simulink model "PFC_DSFB"  (R2023b)
settings: Solver=VariableStepAuto  StartTime=0.0  StopTime=0.5  RelTol=1e-3
libraries: spsVoltageMeasurementLib x5, spsSeriesRLCBranchLib x3, spsCurrentMeasurementLib x3, spsDiodeLib x3, spsMosfetLib x2, spsACVoltageSourceLib x1, simulink x1, spsLinearTransformerLib x1, spsMeanLib x1, slpidlib x1, powerlib_extras x1, simulink_extras x1
settings Model: SimulationMode=accelerator  Creator=abc6820292  LastModifiedBy=Qu
settings DebuggingCC: UnconnectedInputMsg=warning  UnconnectedOutputMsg=warning  UnconnectedLineMsg=warning
settings ModelReferenceCC: EnableRefExpFcnMdlSchedulingChecks=on
settings RTWCC: DLArmComputeVersion=19.05

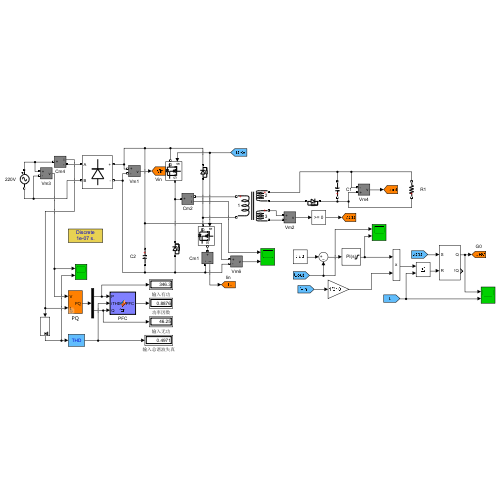
[thumbnail: Simulink's stored preview of the top-level diagram]
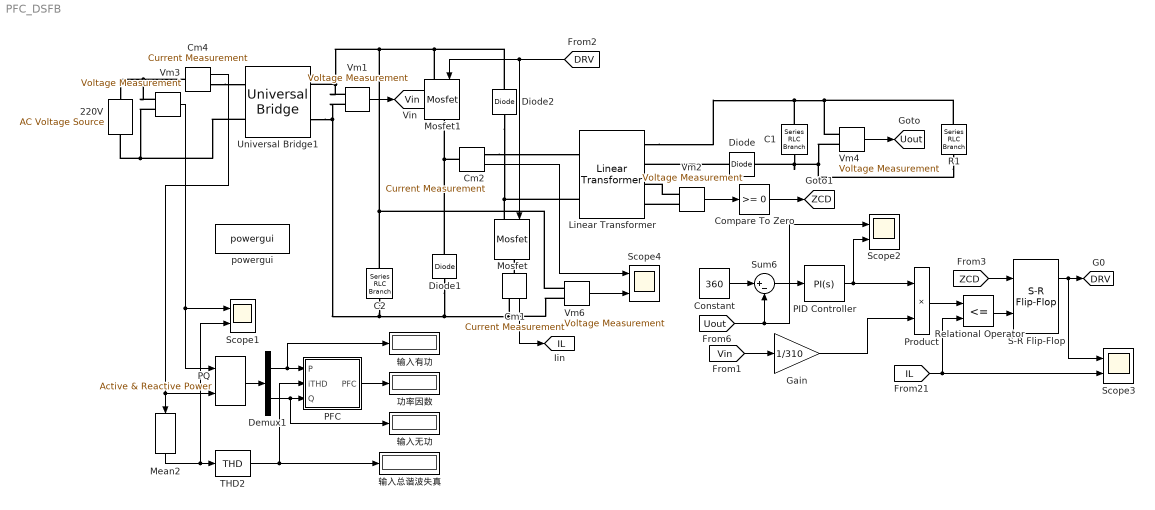
== system PFC_DSFB ==
  220V : spsACVoltageSourceLib/AC Voltage Source  Amplitude=220*1.414  Phase=0  Frequency=50  SampleTime=0  Measurements=None  BusType=swing  Pref=10e3  Qref=0  Qmin=-inf  Qmax=+inf
  C1 : spsSeriesRLCBranchLib/Series RLC Branch  LConnTagsString=__new0  RConnTagsString=__new0  BranchType=C  Resistance=10  Inductance=0  SetiL0=off  InitialCurrent=0  Capacitance=4e-4  Setx0=off  InitialVoltage=200  Measurements=None
  C2 : spsSeriesRLCBranchLib/Series RLC Branch  LConnTagsString=__new0  RConnTagsString=__new0  BranchType=C  Resistance=10  Inductance=0  SetiL0=off  InitialCurrent=0  Capacitance=5e-8  Setx0=off  InitialVoltage=200  Measurements=None
  Cm1 : spsCurrentMeasurementLib/Current Measurement  PhasorSimulation=off  OutputType=Complex  PSBequivalent=0
  Cm2 : spsCurrentMeasurementLib/Current Measurement  PhasorSimulation=off  OutputType=Complex  PSBequivalent=0
  Cm4 : spsCurrentMeasurementLib/Current Measurement  PhasorSimulation=off  OutputType=Complex  PSBequivalent=0
  Compare To Zero : simulink/Logic and Bit Operations/Compare To Zero  relop=>=  OutDataTypeStr=boolean
  Constant : Constant  Value=360
  Demux1 : Demux  Outputs=2
  Diode : spsDiodeLib/Diode  Ron=0.001  Lon=0  Vf=0.8  IC=0  UseSnubber=0  Rs=1e6  Cs=1e-9  Measurements=off
  Diode1 : spsDiodeLib/Diode  Ron=0.001  Lon=0  Vf=0.8  IC=0  UseSnubber=0  Rs=1e6  Cs=1e-9  Measurements=off
  Diode2 : spsDiodeLib/Diode  Ron=0.001  Lon=0  Vf=0.8  IC=0  UseSnubber=0  Rs=1e6  Cs=1e-9  Measurements=off
  Gain : Gain  Gain=1/310
  Linear Transformer : spsLinearTransformerLib/Linear Transformer  UNITS=SI  NominalPower=[600 60000]  winding1=[200 0.01 1e-6]  winding2=[500 0.01 1e-6]  ThreeWindings=on  winding3=[10 1 1e-6]  RmLm=[1e6 2e-4]  Measurements=None  DataType=on
  Mean2 : spsMeanLib/Mean  Freq=2000  Vinit=0  Ts=0
  Mosfet : spsMosfetLib/Mosfet  Ron=0.05  Lon=0  Rd=0.01  Vfd=0  IC=0  Rs=1e5  Cs=inf  Measurements=off
  Mosfet1 : spsMosfetLib/Mosfet  Ron=0.05  Lon=0  Rd=0.01  Vfd=0  IC=0  Rs=1e5  Cs=inf  Measurements=off
  PFC : MATLAB Function  TreatAsAtomicUnit=on
  PID Controller : slpidlib/PID Controller  Controller=PI  Form=Parallel  TimeDomain=Continuous-time  UseExternalTs=off  SampleTime=-1  IntegratorMethod=Forward Euler  FilterMethod=Forward Euler  ControllerParametersSource=internal  P=0.2  I=4  UseKiTs=off  D=0.001  N=100  UseFilter=on  TunerSelectOption=Transfer Function Based (PID Tuner App)  InitialConditionSource=internal  InitialConditionForIntegrator=0  InitialConditionForFilter=0  DifferentiatorICPrevScaledInput=0  ExternalReset=none  TrackingMode=off  Kt=1  LimitOutput=on  SatLimitsSource=internal  UpperSaturationLimit=30  LowerSaturationLimit=0  LinearizeAsGain=on  AntiWindupMode=clamping  Kb=1  LimitIntegrator=off  UpperIntegratorSaturationLimit=inf  LowerIntegratorSaturationLimit=-inf  POutMin=[]  POutMax=[]  IOutMin=[]  IOutMax=[]  DOutMin=[]  DOutMax=[]  NOutMin=[]  NOutMax=[]  SumOutMin=[]  SumOutMax=[]  SaturationOutMin=[]  SaturationOutMax=[]  PParamMin=[]  PParamMax=[]  IParamMin=[]  IParamMax=[]  DParamMin=[]  DParamMax=[]  NParamMin=[]  NParamMax=[]  KbParamMin=[]  KbParamMax=[]  KtParamMin=[]  KtParamMax=[]  KbOutMin=[]  KbOutMax=[]  KtOutMin=[]  KtOutMax=[]  IntegratorOutMin=[]  IntegratorOutMax=[]  FilterOutMin=[]  FilterOutMax=[]  SumI1OutMin=[]  SumI1OutMax=[]  SumI2OutMin=[]  SumI2OutMax=[]  SumI3OutMin=[]  SumI3OutMax=[]  SumI4OutMin=[]  SumI4OutMax=[]  SumDOutMin=[]  SumDOutMax=[]  DifferentiatorOutMin=[]  DifferentiatorOutMax=[]  FilterDiffOutCoefMin=[]  FilterDiffOutCoefMax=[]  ReciprocalOutMin=[]  ReciprocalOutMax=[]  SumDenOutMin=[]  SumDenOutMax=[]  SumNumOutMin=[]  SumNumOutMax=[]  DivideOutMin=[]  DivideOutMax=[]  UdiffTsProdOutMin=[]  UdiffTsProdOutMax=[]  NTsProdOutMin=[]  NTsProdOutMax=[]  UintegralTsProdOutMin=[]  UintegralTsProdOutMax=[]  UngainTsProdOutMin=[]  UngainTsProdOutMax=[]  ClampingZeroOutDataTypeStr=Inherit: Inherit via back propagation  ClampingZeroOutMin=[]  ClampingZeroOutMax=[]  FilterDenConstantOutDataTypeStr=Inherit: Inherit via back propagation  FilterDenConstantOutMin=[]  FilterDenConstantOutMax=[]  PCopyOutDataTypeStr=Inherit: Inherit via back propagation  PCopyOutMin=[]  PCopyOutMax=[]  NCopyOutDataTypeStr=Inherit: Inherit via back propagation  NCopyOutMin=[]  NCopyOutMax=[]  IntegratorContinuousStateAttributes=''  IntegratorStateMustResolveToSignalObject=off  IntegratorRTWStateStorageClass=Auto  FilterContinuousStateAttributes=''  FilterStateMustResolveToSignalObject=off  FilterRTWStateStorageClass=Auto  ParallelPVariant=InternalParameters  IdealPVariant=Disabled  IVariant=InternalParameters  DVariant=Disabled  IntegratorVariant=Continuous  SatVariant=Enabled  AWVariant=ContClampingParallel  PCopyVariant=Disabled  TRVariant=Disabled  FdbkBlocksVariant=Forward  IdealPFdbkVariant=Disabled  SatFdbkVariant=Disabled  DerivativeFilterVariant=Disabled  NVariant=Disabled  NCopyVariant=Disabled_SignalSpec  FilterICVariant=Disabled  IntegratorICVariant=InternalICs  ExternalResetVariant=Disabled  TRSumVariant=Passthrough  SumFdbkVariant=Disabled  SumVariant=Sum_PI  TsampFilterVariant=InternalTs  TsampNgainVariant=Passthrough  TsampIntegralVariant=Disabled_SignalSpec  ExternalSaturationOutDataTypeStr=Inherit: Same as second input
  PQ : powerlib_extras/Measurements/Active & Reactive Power  f1=50
  Product : Product
  R1 : spsSeriesRLCBranchLib/Series RLC Branch  LConnTagsString=__new0  RConnTagsString=__new0  BranchType=R  Resistance=220  Inductance=0  SetiL0=off  InitialCurrent=0  Capacitance=8e-3  Setx0=on  InitialVoltage=280  Measurements=None
  Relational Operator : RelationalOperator  Operator=<=  OutDataTypeStr=boolean  RndMeth=Simplest  InputSameDT=off
  S-R Flip-Flop : simulink_extras/Flip Flops/S-R Flip-Flop  initial_condition=0
  Scope{1..4} (4 alike) : Scope  NumInputPorts=2
  Sum6 : Sum  Inputs=|+-
  THD2 : spsTHDLib/THD  Freq=50  Ts=0
  Universal Bridge1 : spsUniversalBridgeLib/Universal Bridge  Arms=2  SnubberResistance=1e6  SnubberCapacitance=inf  Device=Diodes  Ron=1e-2  Lon=0  ForwardVoltages="[  0  0  ]"  ForwardVoltage=1  GTOparameters=[ 10e-6 , 20e-6 ]  IGBTparameters=[ 1e-6 , 2e-6 ]  Measurements=None  Measurements_2=None  converterType=Rectifier
  Vm{1..4,6} (5 alike) : spsVoltageMeasurementLib/Voltage Measurement  PhasorSimulation=off  OutputType=Complex  PSBequivalent=0
  powergui : spspowerguiLib/powergui  SimulationMode=Discrete  SampleTime=1e-7  frequency=60  Iterations=50  frequencyindice=0  Pbase=100e6  ErrMax=1e-4  UnitsV=kV  UnitsW=MW  buscounter=0  FunctionMessages=off  echomessages=off  EnableUseOfTLC=off  CurrentSourceSwitches=off  DisableSnubberDevices=off  DisableRonSwitches=off  DisableVfSwitches=off  DisplayEquations=off  AutomaticDiscreteSolvers=off  SolverType=Tustin/Backward Euler (TBE)  Interpol=off  ExternalGateDelay=off  methode=off  Ts=0  x0status=blocks  SPID=off  SwTol=0  HookPort=off  NonlinearTolerance=1e-4  nMaxIteration=100  ContinueOnMaxIteration=off  RestoreLinks=warning  ResistiveCurrentMeasurement=off  Frange=[0:2:500]  Ylog=off  Xlog=on  ShowGrid=off  save=off  variable=ZData  structure=QQQQQ  ZoomFFT=off  StartTime=0.5  cycles=15  DisplayStyle=1  fundamental=50  FreqAxis=off  MaxFrequency=1000  frequencyindicesteady=1  RmsSteady=1  display=off
  功率因数 : Display
  输入总谐波失真 : Display
  输入无功 : Display
  输入有功 : Display
  tag scope: DRV=global, IL=global, Uout=global, Vin=global, ZCD=global
  wires:
  Constant/1 -> Sum6/1
  Sum6/1 -> PID Controller/1
  [Uout] -> Scope2/1, Sum6/2
  Vm1/1 -> [Vin]
  PID Controller/1 -> Product/1, Scope2/2
  Vm4/1 -> [Uout]
  Vm2/1 -> Compare To Zero/1
  Compare To Zero/1 -> [ZCD]
  Cm4/1 -> PQ/2, Mean2/1
  [IL] -> Scope3/2, Relational Operator/2
  Demux1/2 -> 输入无功/1, PFC/3(Q)
  Vm3/1 -> Scope1/1, PQ/1
  THD2/1 -> 输入总谐波失真/1, PFC/2(iTHD)
  Demux1/1 -> 输入有功/1, PFC/1(P)
  PFC/1(PFC) -> 功率因数/1
  PQ/1 -> Demux1/1
  Product/1 -> Relational Operator/1
  [Vin] -> Gain/1
  Relational Operator/1 -> S-R Flip-Flop/2
  S-R Flip-Flop/1 -> Scope3/1, [DRV]
  [ZCD] -> S-R Flip-Flop/1
  Vm6/1 -> Scope4/2
  Cm1/1 -> [IL]
  [DRV] -> Mosfet/1, Mosfet1/1
  Cm2/1 -> Scope4/1
  Gain/1 -> Product/2
  Mean2/1 -> Scope1/2, THD2/1
  connections:
  Universal Bridge1/RConn1 -- C2/LConn1 -- Vm6/LConn1 -- Diode2/RConn1 -- Mosfet1/LConn1 -- Vm1/LConn1
  Mosfet/LConn1 -- Linear Transformer/LConn2 -- Diode2/LConn1
  Cm1/LConn1 -- Mosfet/RConn1
  Universal Bridge1/RConn2 -- Vm1/LConn2 -- C2/RConn1 -- Cm1/RConn1 -- Vm6/LConn2 -- Diode1/LConn1
  Vm2/LConn2 -- Linear Transformer/RConn4
  Vm2/LConn1 -- Linear Transformer/RConn3
  Cm4/RConn1 -- Universal Bridge1/LConn1
  Cm4/LConn1 -- Vm3/LConn1 -- 220V/RConn1
  Vm3/LConn2 -- 220V/LConn1 -- Universal Bridge1/LConn2
  Diode/LConn1 -- Linear Transformer/RConn2
  C1/LConn1 -- Vm4/LConn1 -- R1/LConn1 -- Diode/RConn1
  C1/RConn1 -- R1/RConn1 -- Vm4/LConn2 -- Linear Transformer/RConn1
  Diode1/RConn1 -- Cm2/LConn1 -- Mosfet1/RConn1
  Cm2/RConn1 -- Linear Transformer/LConn1

== matlab function PFC_DSFB/PFC ==
  data: P input; iTHD input; PFC output; Q input
function PFC = fcn(P,iTHD,Q)
% This block supports an embeddable subset of the MATLAB language.
% See the help menu for details. 
PFC=(P/sqrt(P*P+Q*Q))/sqrt(1+iTHD*iTHD);
